simulink model "PFCnew"  (R2024b)
settings: Solver=VariableStepAuto  StartTime=0.0  StopTime=0.1  RelTol=1e-3
libraries: spsSeriesRLCBranchLib x4, spsVoltageMeasurementLib x3, spsCurrentMeasurementLib x2, spsACVoltageSourceLib x1, spsDiodeLib x1, spsIdealSwitchLib x1, spsMosfetLib x1, spsPWMGeneratorDCDCLib x1, spsUniversalBridgeLib x1, sps_lib x1
settings Model: Creator=Asus  LastModifiedBy=Asus

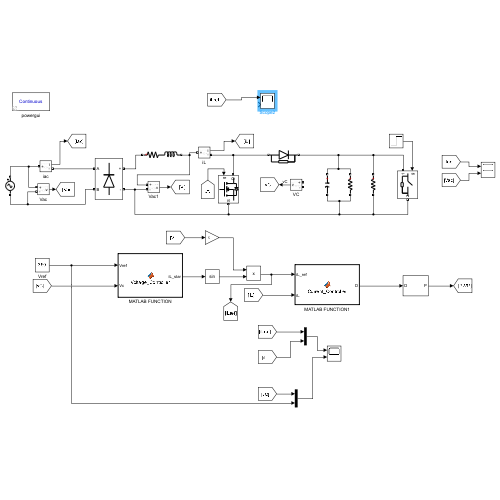
[thumbnail: Simulink's stored preview of the top-level diagram]
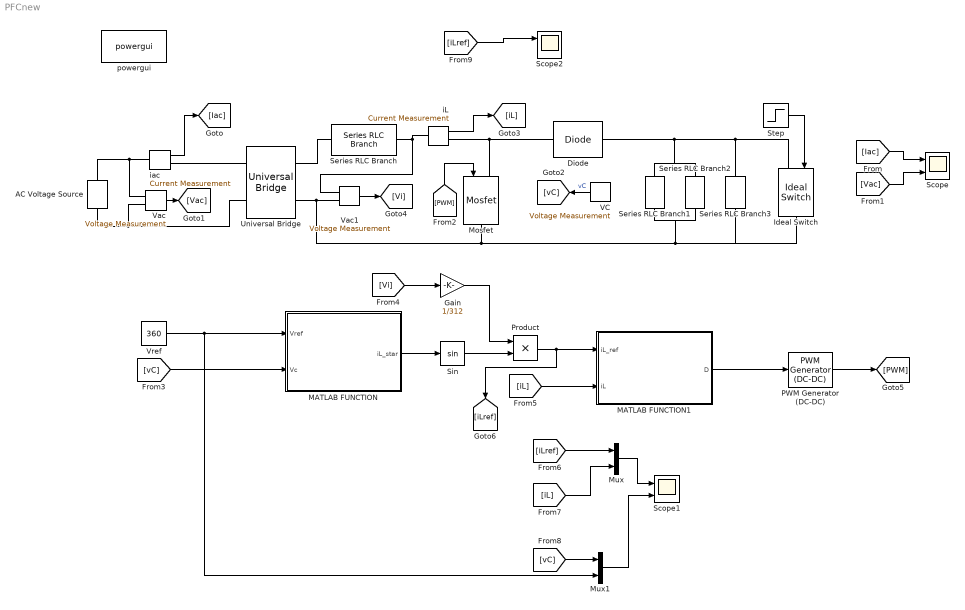
== system PFCnew ==
  AC Voltage Source : spsACVoltageSourceLib/AC Voltage Source  Amplitude=312  Phase=0  Frequency=50  SampleTime=0  Measurements=None  BusType=swing  Pref=10e3  Qref=0  Qmin=-inf  Qmax=+inf
  Diode : spsDiodeLib/Diode  Ron=0.001  Lon=0  Vf=0.8  IC=0  UseSnubber=0  Rs=500  Cs=250e-9  Measurements=off
  Gain : Gain  Gain=1/312
  Ideal Switch : spsIdealSwitchLib/Ideal Switch  Ron=0.001  Lon=0  IC=0  Rs=1e5  Cs=inf  Measurements=off
  MATLAB FUNCTION : MATLAB Function  TreatAsAtomicUnit=on
  MATLAB FUNCTION1 : MATLAB Function  TreatAsAtomicUnit=on
  Mosfet : spsMosfetLib/Mosfet  Ron=0.1  Lon=0  Rd=0.01  Vfd=0  IC=0  Rs=1e5  Cs=inf  Measurements=off
  Mux : Mux  Inputs=2
  Mux1 : Mux  Inputs=2
  PWM Generator (DC-DC) : spsPWMGeneratorDCDCLib/PWM Generator (DC-DC)  Fsw=30000  Ts=0
  Product : Product
  Scope : Scope  NumInputPorts=2
  Scope1 : Scope  NumInputPorts=2
  Scope2 : Scope  NumInputPorts=2
  Series RLC Branch : spsSeriesRLCBranchLib/Series RLC Branch  LConnTagsString=__new0  RConnTagsString=__new0  BranchType=RL  Resistance=0.05  Inductance=2e-3  SetiL0=off  InitialCurrent=0  Capacitance=1e-6  Setx0=off  InitialVoltage=0  Measurements=None
  Series RLC Branch1 : spsSeriesRLCBranchLib/Series RLC Branch  LConnTagsString=__new0  RConnTagsString=__new0  BranchType=C  Resistance=0.05  Inductance=2e-3  SetiL0=off  InitialCurrent=0  Capacitance=2200e-6  Setx0=off  InitialVoltage=0  Measurements=None
  Series RLC Branch2 : spsSeriesRLCBranchLib/Series RLC Branch  LConnTagsString=__new0  RConnTagsString=__new0  BranchType=R  Resistance=180  Inductance=2e-3  SetiL0=off  InitialCurrent=0  Capacitance=1e-6  Setx0=off  InitialVoltage=0  Measurements=None
  Series RLC Branch3 : spsSeriesRLCBranchLib/Series RLC Branch  LConnTagsString=__new0  RConnTagsString=__new0  BranchType=R  Resistance=1  Inductance=2e-3  SetiL0=off  InitialCurrent=0  Capacitance=1e-6  Setx0=off  InitialVoltage=0  Measurements=None
  Sin : Trigonometry
  Step : Step  SampleTime=0
  Universal Bridge : spsUniversalBridgeLib/Universal Bridge  Arms=2  SnubberResistance=1e5  SnubberCapacitance=inf  Device=Diodes  Ron=1e-3  Lon=0  ForwardVoltages="[  0  0  ]"  ForwardVoltage=0  GTOparameters=[ 10e-6 , 20e-6 ]  IGBTparameters=[ 1e-6 , 2e-6 ]  Measurements=None  Measurements_2=None  converterType=Rectifier
  VC : spsVoltageMeasurementLib/Voltage Measurement  PhasorSimulation=off  OutputType=Complex  PSBequivalent=0
  Vac : spsVoltageMeasurementLib/Voltage Measurement  PhasorSimulation=off  OutputType=Complex  PSBequivalent=0
  Vac1 : spsVoltageMeasurementLib/Voltage Measurement  PhasorSimulation=off  OutputType=Complex  PSBequivalent=0
  Vref : Constant  Value=360
  iL : spsCurrentMeasurementLib/Current Measurement  PhasorSimulation=off  OutputType=Complex  PSBequivalent=0
  iac : spsCurrentMeasurementLib/Current Measurement  PhasorSimulation=off  OutputType=Complex  PSBequivalent=0
  powergui : sps_lib/powergui  Priority=1  SimulationMode=Continuous  SampleTime=50e-6  frequency=60  Iterations=50  frequencyindice=50  Pbase=100e6  ErrMax=1e-4  UnitsV=kV  UnitsW=MW  buscounter=0  FunctionMessages=off  echomessages=off  EnableUseOfTLC=off  CurrentSourceSwitches=off  DisableSnubberDevices=off  DisableRonSwitches=off  DisableVfSwitches=off  DisplayEquations=off  AutomaticDiscreteSolvers=off  SolverType=Tustin/Backward Euler (TBE)  Interpol=off  ExternalGateDelay=off  methode=off  Ts=100  x0status=blocks  SPID=on  SwTol=0  HookPort=off  NonlinearTolerance=1e-4  nMaxIteration=100  ContinueOnMaxIteration=off  RestoreLinks=warning  ResistiveCurrentMeasurement=off  Frange=[0:2:500]  Ylog=off  Xlog=on  ShowGrid=off  save=off  variable=ZData  structure=0  ZoomFFT=off  StartTime=0.0  cycles=1  DisplayStyle=1  fundamental=60  FreqAxis=off  MaxFrequency=1000  frequencyindicesteady=1  RmsSteady=1  display=off
  wires:
  Step/1 -> Ideal Switch/1
  iac/1 -> [Iac]
  Vac/1 -> [Vac]
  [Iac] -> Scope/1
  [Vac] -> Scope/2
  [PWM] -> Mosfet/1
  VC/1 -> [vC]  "vC"
  iL/1 -> [iL]
  Vref/1 -> Mux1/2, MATLAB FUNCTION/1(Vref)
  [vC] -> MATLAB FUNCTION/2(Vc)
  Vac1/1 -> [Vi]
  [Vi] -> Gain/1
  Gain/1 -> Product/1
  Product/1 -> [iLref], MATLAB FUNCTION1/1(iL_ref)
  MATLAB FUNCTION1/1(D) -> PWM Generator (DC-DC)/1
  PWM Generator (DC-DC)/1 -> [PWM]
  [iL] -> MATLAB FUNCTION1/2(iL)
  [iLref] -> Mux/1
  [iL] -> Mux/2
  Mux/1 -> Scope1/1
  [vC] -> Mux1/1
  Mux1/1 -> Scope1/2
  [iLref] -> Scope2/1
  MATLAB FUNCTION/1(iL_star) -> Sin/1
  Sin/1 -> Product/2
  connections:
  Universal Bridge/RConn1 -- Series RLC Branch/LConn1
  Mosfet/LConn1 -- Diode/LConn1 -- iL/RConn1
  Series RLC Branch/RConn1 -- iL/LConn1 -- Vac1/LConn1
  Diode/RConn1 -- Series RLC Branch1/LConn1 -- Series RLC Branch2/LConn1 -- Ideal Switch/LConn1 -- Series RLC Branch3/LConn1
  Universal Bridge/RConn2 -- Ideal Switch/RConn1 -- Series RLC Branch3/RConn1 -- Series RLC Branch1/RConn1 -- Series RLC Branch2/RConn1 -- Mosfet/RConn1 -- Vac1/LConn2
  AC Voltage Source/LConn1 -- Universal Bridge/LConn2 -- Vac/LConn2
  iac/RConn1 -- Universal Bridge/LConn1
  AC Voltage Source/RConn1 -- Vac/LConn1 -- iac/LConn1

== matlab function PFCnew/MATLAB FUNCTION ==
  settings: updateMethod=DISCRETE
  data: iL_star output; Vref input; Vc input
function iL_star = Voltage_Controller(Vref,Vc)


Kp = 0.1293;
Ki = 4.06;


Ts = 1/30000;

persistent integral

if isempty(integral)
    integral = 0;
end

error_v = Vref - Vc;

integral = integral + error_v*Ts;

iL_star = Kp*error_v + Ki*integral;

end

== matlab function PFCnew/MATLAB FUNCTION1 ==
  settings: updateMethod=DISCRETE
  data: D output; iL_ref input; iL input
function D = Current_Controller(iL_ref,iL)

Kp = 0.0154397;
Ki = 22.2551;


Ts = 1/30000;

persistent integral

if isempty(integral)
    integral = 0;
end


error_i = iL_ref - iL;


integral = integral + error_i*Ts;


D = Kp*error_i + Ki*integral;

if D > 0.95
    D = 0.95;
elseif D < 0
    D = 0;
end

end
